simulink model "r2_b8a4x1kf"  (R2012b)
settings: Solver=VariableStepDiscrete  SolverMode=SingleTasking  StartTime=0.0  StopTime=1  RelTol=1e-3
undefined symbols (not defined in the file): fft_stages, n_bits_ants, n_bits_xengs
libraries: xbsIndex_r4 x22142, casper_library_misc x166, xbsReplacements_r4 x24, casper_library_delays x8, xps_library x5, casper_library_communications x4
(part 120 of 178)

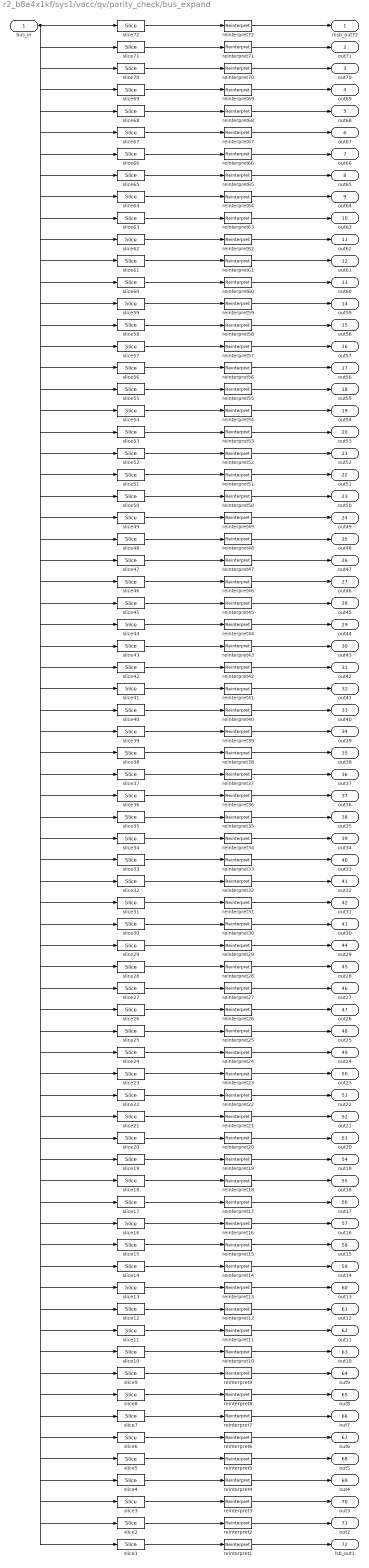
== system r2_b8a4x1kf/sys1/vacc/qv/parity_check/bus_expand ==
  bus_in : Inport
  reinterpret{1..72} (72 alike) : xbsIndex_r4/Reinterpret  force_arith_type=on  arith_type=Unsigned  force_bin_pt=on  bin_pt=0  block_type=reinterpret
  slice1 : xbsIndex_r4/Slice  nbits=1  boolean_output=off  mode=Upper Bit Location + Width  bit1=-71  base1=MSB of Input  bit0=0  base0=LSB of Input  dbl_ovrd=off  block_type=slice
  slice10 : xbsIndex_r4/Slice  nbits=1  boolean_output=off  mode=Upper Bit Location + Width  bit1=-62  base1=MSB of Input  bit0=0  base0=LSB of Input  dbl_ovrd=off  block_type=slice
  slice11 : xbsIndex_r4/Slice  nbits=1  boolean_output=off  mode=Upper Bit Location + Width  bit1=-61  base1=MSB of Input  bit0=0  base0=LSB of Input  dbl_ovrd=off  block_type=slice
  slice12 : xbsIndex_r4/Slice  nbits=1  boolean_output=off  mode=Upper Bit Location + Width  bit1=-60  base1=MSB of Input  bit0=0  base0=LSB of Input  dbl_ovrd=off  block_type=slice
  slice13 : xbsIndex_r4/Slice  nbits=1  boolean_output=off  mode=Upper Bit Location + Width  bit1=-59  base1=MSB of Input  bit0=0  base0=LSB of Input  dbl_ovrd=off  block_type=slice
  slice14 : xbsIndex_r4/Slice  nbits=1  boolean_output=off  mode=Upper Bit Location + Width  bit1=-58  base1=MSB of Input  bit0=0  base0=LSB of Input  dbl_ovrd=off  block_type=slice
  slice15 : xbsIndex_r4/Slice  nbits=1  boolean_output=off  mode=Upper Bit Location + Width  bit1=-57  base1=MSB of Input  bit0=0  base0=LSB of Input  dbl_ovrd=off  block_type=slice
  slice16 : xbsIndex_r4/Slice  nbits=1  boolean_output=off  mode=Upper Bit Location + Width  bit1=-56  base1=MSB of Input  bit0=0  base0=LSB of Input  dbl_ovrd=off  block_type=slice
  slice17 : xbsIndex_r4/Slice  nbits=1  boolean_output=off  mode=Upper Bit Location + Width  bit1=-55  base1=MSB of Input  bit0=0  base0=LSB of Input  dbl_ovrd=off  block_type=slice
  slice18 : xbsIndex_r4/Slice  nbits=1  boolean_output=off  mode=Upper Bit Location + Width  bit1=-54  base1=MSB of Input  bit0=0  base0=LSB of Input  dbl_ovrd=off  block_type=slice
  slice19 : xbsIndex_r4/Slice  nbits=1  boolean_output=off  mode=Upper Bit Location + Width  bit1=-53  base1=MSB of Input  bit0=0  base0=LSB of Input  dbl_ovrd=off  block_type=slice
  slice2 : xbsIndex_r4/Slice  nbits=1  boolean_output=off  mode=Upper Bit Location + Width  bit1=-70  base1=MSB of Input  bit0=0  base0=LSB of Input  dbl_ovrd=off  block_type=slice
  slice20 : xbsIndex_r4/Slice  nbits=1  boolean_output=off  mode=Upper Bit Location + Width  bit1=-52  base1=MSB of Input  bit0=0  base0=LSB of Input  dbl_ovrd=off  block_type=slice
  slice21 : xbsIndex_r4/Slice  nbits=1  boolean_output=off  mode=Upper Bit Location + Width  bit1=-51  base1=MSB of Input  bit0=0  base0=LSB of Input  dbl_ovrd=off  block_type=slice
  slice22 : xbsIndex_r4/Slice  nbits=1  boolean_output=off  mode=Upper Bit Location + Width  bit1=-50  base1=MSB of Input  bit0=0  base0=LSB of Input  dbl_ovrd=off  block_type=slice
  slice23 : xbsIndex_r4/Slice  nbits=1  boolean_output=off  mode=Upper Bit Location + Width  bit1=-49  base1=MSB of Input  bit0=0  base0=LSB of Input  dbl_ovrd=off  block_type=slice
  slice24 : xbsIndex_r4/Slice  nbits=1  boolean_output=off  mode=Upper Bit Location + Width  bit1=-48  base1=MSB of Input  bit0=0  base0=LSB of Input  dbl_ovrd=off  block_type=slice
  slice25 : xbsIndex_r4/Slice  nbits=1  boolean_output=off  mode=Upper Bit Location + Width  bit1=-47  base1=MSB of Input  bit0=0  base0=LSB of Input  dbl_ovrd=off  block_type=slice
  slice26 : xbsIndex_r4/Slice  nbits=1  boolean_output=off  mode=Upper Bit Location + Width  bit1=-46  base1=MSB of Input  bit0=0  base0=LSB of Input  dbl_ovrd=off  block_type=slice
  slice27 : xbsIndex_r4/Slice  nbits=1  boolean_output=off  mode=Upper Bit Location + Width  bit1=-45  base1=MSB of Input  bit0=0  base0=LSB of Input  dbl_ovrd=off  block_type=slice
  slice28 : xbsIndex_r4/Slice  nbits=1  boolean_output=off  mode=Upper Bit Location + Width  bit1=-44  base1=MSB of Input  bit0=0  base0=LSB of Input  dbl_ovrd=off  block_type=slice
  slice29 : xbsIndex_r4/Slice  nbits=1  boolean_output=off  mode=Upper Bit Location + Width  bit1=-43  base1=MSB of Input  bit0=0  base0=LSB of Input  dbl_ovrd=off  block_type=slice
  slice3 : xbsIndex_r4/Slice  nbits=1  boolean_output=off  mode=Upper Bit Location + Width  bit1=-69  base1=MSB of Input  bit0=0  base0=LSB of Input  dbl_ovrd=off  block_type=slice
  slice30 : xbsIndex_r4/Slice  nbits=1  boolean_output=off  mode=Upper Bit Location + Width  bit1=-42  base1=MSB of Input  bit0=0  base0=LSB of Input  dbl_ovrd=off  block_type=slice
  slice31 : xbsIndex_r4/Slice  nbits=1  boolean_output=off  mode=Upper Bit Location + Width  bit1=-41  base1=MSB of Input  bit0=0  base0=LSB of Input  dbl_ovrd=off  block_type=slice
  slice32 : xbsIndex_r4/Slice  nbits=1  boolean_output=off  mode=Upper Bit Location + Width  bit1=-40  base1=MSB of Input  bit0=0  base0=LSB of Input  dbl_ovrd=off  block_type=slice
  slice33 : xbsIndex_r4/Slice  nbits=1  boolean_output=off  mode=Upper Bit Location + Width  bit1=-39  base1=MSB of Input  bit0=0  base0=LSB of Input  dbl_ovrd=off  block_type=slice
  slice34 : xbsIndex_r4/Slice  nbits=1  boolean_output=off  mode=Upper Bit Location + Width  bit1=-38  base1=MSB of Input  bit0=0  base0=LSB of Input  dbl_ovrd=off  block_type=slice
  slice35 : xbsIndex_r4/Slice  nbits=1  boolean_output=off  mode=Upper Bit Location + Width  bit1=-37  base1=MSB of Input  bit0=0  base0=LSB of Input  dbl_ovrd=off  block_type=slice
  slice36 : xbsIndex_r4/Slice  nbits=1  boolean_output=off  mode=Upper Bit Location + Width  bit1=-36  base1=MSB of Input  bit0=0  base0=LSB of Input  dbl_ovrd=off  block_type=slice
  slice37 : xbsIndex_r4/Slice  nbits=1  boolean_output=off  mode=Upper Bit Location + Width  bit1=-35  base1=MSB of Input  bit0=0  base0=LSB of Input  dbl_ovrd=off  block_type=slice
  slice38 : xbsIndex_r4/Slice  nbits=1  boolean_output=off  mode=Upper Bit Location + Width  bit1=-34  base1=MSB of Input  bit0=0  base0=LSB of Input  dbl_ovrd=off  block_type=slice
  slice39 : xbsIndex_r4/Slice  nbits=1  boolean_output=off  mode=Upper Bit Location + Width  bit1=-33  base1=MSB of Input  bit0=0  base0=LSB of Input  dbl_ovrd=off  block_type=slice
  slice4 : xbsIndex_r4/Slice  nbits=1  boolean_output=off  mode=Upper Bit Location + Width  bit1=-68  base1=MSB of Input  bit0=0  base0=LSB of Input  dbl_ovrd=off  block_type=slice
  slice40 : xbsIndex_r4/Slice  nbits=1  boolean_output=off  mode=Upper Bit Location + Width  bit1=-32  base1=MSB of Input  bit0=0  base0=LSB of Input  dbl_ovrd=off  block_type=slice
  slice41 : xbsIndex_r4/Slice  nbits=1  boolean_output=off  mode=Upper Bit Location + Width  bit1=-31  base1=MSB of Input  bit0=0  base0=LSB of Input  dbl_ovrd=off  block_type=slice
  slice42 : xbsIndex_r4/Slice  nbits=1  boolean_output=off  mode=Upper Bit Location + Width  bit1=-30  base1=MSB of Input  bit0=0  base0=LSB of Input  dbl_ovrd=off  block_type=slice
  slice43 : xbsIndex_r4/Slice  nbits=1  boolean_output=off  mode=Upper Bit Location + Width  bit1=-29  base1=MSB of Input  bit0=0  base0=LSB of Input  dbl_ovrd=off  block_type=slice
  slice44 : xbsIndex_r4/Slice  nbits=1  boolean_output=off  mode=Upper Bit Location + Width  bit1=-28  base1=MSB of Input  bit0=0  base0=LSB of Input  dbl_ovrd=off  block_type=slice
  slice45 : xbsIndex_r4/Slice  nbits=1  boolean_output=off  mode=Upper Bit Location + Width  bit1=-27  base1=MSB of Input  bit0=0  base0=LSB of Input  dbl_ovrd=off  block_type=slice
  slice46 : xbsIndex_r4/Slice  nbits=1  boolean_output=off  mode=Upper Bit Location + Width  bit1=-26  base1=MSB of Input  bit0=0  base0=LSB of Input  dbl_ovrd=off  block_type=slice
  slice47 : xbsIndex_r4/Slice  nbits=1  boolean_output=off  mode=Upper Bit Location + Width  bit1=-25  base1=MSB of Input  bit0=0  base0=LSB of Input  dbl_ovrd=off  block_type=slice
  slice48 : xbsIndex_r4/Slice  nbits=1  boolean_output=off  mode=Upper Bit Location + Width  bit1=-24  base1=MSB of Input  bit0=0  base0=LSB of Input  dbl_ovrd=off  block_type=slice
  slice49 : xbsIndex_r4/Slice  nbits=1  boolean_output=off  mode=Upper Bit Location + Width  bit1=-23  base1=MSB of Input  bit0=0  base0=LSB of Input  dbl_ovrd=off  block_type=slice
  slice5 : xbsIndex_r4/Slice  nbits=1  boolean_output=off  mode=Upper Bit Location + Width  bit1=-67  base1=MSB of Input  bit0=0  base0=LSB of Input  dbl_ovrd=off  block_type=slice
  slice50 : xbsIndex_r4/Slice  nbits=1  boolean_output=off  mode=Upper Bit Location + Width  bit1=-22  base1=MSB of Input  bit0=0  base0=LSB of Input  dbl_ovrd=off  block_type=slice
  slice51 : xbsIndex_r4/Slice  nbits=1  boolean_output=off  mode=Upper Bit Location + Width  bit1=-21  base1=MSB of Input  bit0=0  base0=LSB of Input  dbl_ovrd=off  block_type=slice
  slice52 : xbsIndex_r4/Slice  nbits=1  boolean_output=off  mode=Upper Bit Location + Width  bit1=-20  base1=MSB of Input  bit0=0  base0=LSB of Input  dbl_ovrd=off  block_type=slice
  slice53 : xbsIndex_r4/Slice  nbits=1  boolean_output=off  mode=Upper Bit Location + Width  bit1=-19  base1=MSB of Input  bit0=0  base0=LSB of Input  dbl_ovrd=off  block_type=slice
  slice54 : xbsIndex_r4/Slice  nbits=1  boolean_output=off  mode=Upper Bit Location + Width  bit1=-18  base1=MSB of Input  bit0=0  base0=LSB of Input  dbl_ovrd=off  block_type=slice
  slice55 : xbsIndex_r4/Slice  nbits=1  boolean_output=off  mode=Upper Bit Location + Width  bit1=-17  base1=MSB of Input  bit0=0  base0=LSB of Input  dbl_ovrd=off  block_type=slice
  slice56 : xbsIndex_r4/Slice  nbits=1  boolean_output=off  mode=Upper Bit Location + Width  bit1=-16  base1=MSB of Input  bit0=0  base0=LSB of Input  dbl_ovrd=off  block_type=slice
  slice57 : xbsIndex_r4/Slice  nbits=1  boolean_output=off  mode=Upper Bit Location + Width  bit1=-15  base1=MSB of Input  bit0=0  base0=LSB of Input  dbl_ovrd=off  block_type=slice
  slice58 : xbsIndex_r4/Slice  nbits=1  boolean_output=off  mode=Upper Bit Location + Width  bit1=-14  base1=MSB of Input  bit0=0  base0=LSB of Input  dbl_ovrd=off  block_type=slice
  slice59 : xbsIndex_r4/Slice  nbits=1  boolean_output=off  mode=Upper Bit Location + Width  bit1=-13  base1=MSB of Input  bit0=0  base0=LSB of Input  dbl_ovrd=off  block_type=slice
  slice6 : xbsIndex_r4/Slice  nbits=1  boolean_output=off  mode=Upper Bit Location + Width  bit1=-66  base1=MSB of Input  bit0=0  base0=LSB of Input  dbl_ovrd=off  block_type=slice
  slice60 : xbsIndex_r4/Slice  nbits=1  boolean_output=off  mode=Upper Bit Location + Width  bit1=-12  base1=MSB of Input  bit0=0  base0=LSB of Input  dbl_ovrd=off  block_type=slice
  slice61 : xbsIndex_r4/Slice  nbits=1  boolean_output=off  mode=Upper Bit Location + Width  bit1=-11  base1=MSB of Input  bit0=0  base0=LSB of Input  dbl_ovrd=off  block_type=slice
  slice62 : xbsIndex_r4/Slice  nbits=1  boolean_output=off  mode=Upper Bit Location + Width  bit1=-10  base1=MSB of Input  bit0=0  base0=LSB of Input  dbl_ovrd=off  block_type=slice
  slice63 : xbsIndex_r4/Slice  nbits=1  boolean_output=off  mode=Upper Bit Location + Width  bit1=-9  base1=MSB of Input  bit0=0  base0=LSB of Input  dbl_ovrd=off  block_type=slice
  slice64 : xbsIndex_r4/Slice  nbits=1  boolean_output=off  mode=Upper Bit Location + Width  bit1=-8  base1=MSB of Input  bit0=0  base0=LSB of Input  dbl_ovrd=off  block_type=slice
  slice65 : xbsIndex_r4/Slice  nbits=1  boolean_output=off  mode=Upper Bit Location + Width  bit1=-7  base1=MSB of Input  bit0=0  base0=LSB of Input  dbl_ovrd=off  block_type=slice
  slice66 : xbsIndex_r4/Slice  nbits=1  boolean_output=off  mode=Upper Bit Location + Width  bit1=-6  base1=MSB of Input  bit0=0  base0=LSB of Input  dbl_ovrd=off  block_type=slice
  slice67 : xbsIndex_r4/Slice  nbits=1  boolean_output=off  mode=Upper Bit Location + Width  bit1=-5  base1=MSB of Input  bit0=0  base0=LSB of Input  dbl_ovrd=off  block_type=slice
  slice68 : xbsIndex_r4/Slice  nbits=1  boolean_output=off  mode=Upper Bit Location + Width  bit1=-4  base1=MSB of Input  bit0=0  base0=LSB of Input  dbl_ovrd=off  block_type=slice
  slice69 : xbsIndex_r4/Slice  nbits=1  boolean_output=off  mode=Upper Bit Location + Width  bit1=-3  base1=MSB of Input  bit0=0  base0=LSB of Input  dbl_ovrd=off  block_type=slice
  slice7 : xbsIndex_r4/Slice  nbits=1  boolean_output=off  mode=Upper Bit Location + Width  bit1=-65  base1=MSB of Input  bit0=0  base0=LSB of Input  dbl_ovrd=off  block_type=slice
  slice70 : xbsIndex_r4/Slice  nbits=1  boolean_output=off  mode=Upper Bit Location + Width  bit1=-2  base1=MSB of Input  bit0=0  base0=LSB of Input  dbl_ovrd=off  block_type=slice
  slice71 : xbsIndex_r4/Slice  nbits=1  boolean_output=off  mode=Upper Bit Location + Width  bit1=-1  base1=MSB of Input  bit0=0  base0=LSB of Input  dbl_ovrd=off  block_type=slice
  slice72 : xbsIndex_r4/Slice  nbits=1  boolean_output=off  mode=Upper Bit Location + Width  bit1=0  base1=MSB of Input  bit0=0  base0=LSB of Input  dbl_ovrd=off  block_type=slice
  slice8 : xbsIndex_r4/Slice  nbits=1  boolean_output=off  mode=Upper Bit Location + Width  bit1=-64  base1=MSB of Input  bit0=0  base0=LSB of Input  dbl_ovrd=off  block_type=slice
  slice9 : xbsIndex_r4/Slice  nbits=1  boolean_output=off  mode=Upper Bit Location + Width  bit1=-63  base1=MSB of Input  bit0=0  base0=LSB of Input  dbl_ovrd=off  block_type=slice
  msb_out72 : Outport
  out71 : Outport  Port=2
  out70 : Outport  Port=3
  out69 : Outport  Port=4
  out68 : Outport  Port=5
  out67 : Outport  Port=6
  out66 : Outport  Port=7
  out65 : Outport  Port=8
  out64 : Outport  Port=9
  out63 : Outport  Port=10
  out62 : Outport  Port=11
  out61 : Outport  Port=12
  out60 : Outport  Port=13
  out59 : Outport  Port=14
  out58 : Outport  Port=15
  out57 : Outport  Port=16
  out56 : Outport  Port=17
  out55 : Outport  Port=18
  out54 : Outport  Port=19
  out53 : Outport  Port=20
  out52 : Outport  Port=21
  out51 : Outport  Port=22
  out50 : Outport  Port=23
  out49 : Outport  Port=24
  out48 : Outport  Port=25
  out47 : Outport  Port=26
  out46 : Outport  Port=27
  out45 : Outport  Port=28
  out44 : Outport  Port=29
  out43 : Outport  Port=30
  out42 : Outport  Port=31
  out41 : Outport  Port=32
  out40 : Outport  Port=33
  out39 : Outport  Port=34
  out38 : Outport  Port=35
  out37 : Outport  Port=36
  out36 : Outport  Port=37
  out35 : Outport  Port=38
  out34 : Outport  Port=39
  out33 : Outport  Port=40
  out32 : Outport  Port=41
  out31 : Outport  Port=42
  out30 : Outport  Port=43
  out29 : Outport  Port=44
  out28 : Outport  Port=45
  out27 : Outport  Port=46
  out26 : Outport  Port=47
  out25 : Outport  Port=48
  out24 : Outport  Port=49
  out23 : Outport  Port=50
  out22 : Outport  Port=51
  out21 : Outport  Port=52
  out20 : Outport  Port=53
  out19 : Outport  Port=54
  out18 : Outport  Port=55
  out17 : Outport  Port=56
  out16 : Outport  Port=57
  out15 : Outport  Port=58
  out14 : Outport  Port=59
  out13 : Outport  Port=60
  out12 : Outport  Port=61
  out11 : Outport  Port=62
  out10 : Outport  Port=63
  out9 : Outport  Port=64
  out8 : Outport  Port=65
  out7 : Outport  Port=66
  out6 : Outport  Port=67
  out5 : Outport  Port=68
  out4 : Outport  Port=69
  out3 : Outport  Port=70
  out2 : Outport  Port=71
  lsb_out1 : Outport  Port=72
  wires:
  reinterpret1/1 -> lsb_out1/1
  slice1/1 -> reinterpret1/1
  reinterpret2/1 -> out2/1
  slice2/1 -> reinterpret2/1
  reinterpret3/1 -> out3/1
  slice3/1 -> reinterpret3/1
  reinterpret4/1 -> out4/1
  slice4/1 -> reinterpret4/1
  reinterpret5/1 -> out5/1
  slice5/1 -> reinterpret5/1
  reinterpret6/1 -> out6/1
  slice6/1 -> reinterpret6/1
  reinterpret7/1 -> out7/1
  slice7/1 -> reinterpret7/1
  reinterpret8/1 -> out8/1
  slice8/1 -> reinterpret8/1
  reinterpret9/1 -> out9/1
  slice9/1 -> reinterpret9/1
  reinterpret10/1 -> out10/1
  slice10/1 -> reinterpret10/1
  reinterpret11/1 -> out11/1
  slice11/1 -> reinterpret11/1
  reinterpret12/1 -> out12/1
  slice12/1 -> reinterpret12/1
  reinterpret13/1 -> out13/1
  slice13/1 -> reinterpret13/1
  reinterpret14/1 -> out14/1
  slice14/1 -> reinterpret14/1
  reinterpret15/1 -> out15/1
  slice15/1 -> reinterpret15/1
  reinterpret16/1 -> out16/1
  slice16/1 -> reinterpret16/1
  reinterpret17/1 -> out17/1
  slice17/1 -> reinterpret17/1
  reinterpret18/1 -> out18/1
  slice18/1 -> reinterpret18/1
  reinterpret19/1 -> out19/1
  slice19/1 -> reinterpret19/1
  reinterpret20/1 -> out20/1
  slice20/1 -> reinterpret20/1
  reinterpret21/1 -> out21/1
  slice21/1 -> reinterpret21/1
  reinterpret22/1 -> out22/1
  slice22/1 -> reinterpret22/1
  reinterpret23/1 -> out23/1
  slice23/1 -> reinterpret23/1
  reinterpret24/1 -> out24/1
  slice24/1 -> reinterpret24/1
  reinterpret25/1 -> out25/1
  slice25/1 -> reinterpret25/1
  reinterpret26/1 -> out26/1
  slice26/1 -> reinterpret26/1
  reinterpret27/1 -> out27/1
  slice27/1 -> reinterpret27/1
  reinterpret28/1 -> out28/1
  slice28/1 -> reinterpret28/1
  reinterpret29/1 -> out29/1
  slice29/1 -> reinterpret29/1
  reinterpret30/1 -> out30/1
  slice30/1 -> reinterpret30/1
  reinterpret31/1 -> out31/1
  slice31/1 -> reinterpret31/1
  reinterpret32/1 -> out32/1
  slice32/1 -> reinterpret32/1
  reinterpret33/1 -> out33/1
  slice33/1 -> reinterpret33/1
  reinterpret34/1 -> out34/1
  slice34/1 -> reinterpret34/1
  reinterpret35/1 -> out35/1
  slice35/1 -> reinterpret35/1
  reinterpret36/1 -> out36/1
  slice36/1 -> reinterpret36/1
  reinterpret37/1 -> out37/1
  slice37/1 -> reinterpret37/1
  reinterpret38/1 -> out38/1
  slice38/1 -> reinterpret38/1
  reinterpret39/1 -> out39/1
  slice39/1 -> reinterpret39/1
  reinterpret40/1 -> out40/1
  slice40/1 -> reinterpret40/1
  reinterpret41/1 -> out41/1
  slice41/1 -> reinterpret41/1
  reinterpret42/1 -> out42/1
  slice42/1 -> reinterpret42/1
  reinterpret43/1 -> out43/1
  slice43/1 -> reinterpret43/1
  reinterpret44/1 -> out44/1
  slice44/1 -> reinterpret44/1
  reinterpret45/1 -> out45/1
  slice45/1 -> reinterpret45/1
  reinterpret46/1 -> out46/1
  slice46/1 -> reinterpret46/1
  reinterpret47/1 -> out47/1
  slice47/1 -> reinterpret47/1
  reinterpret48/1 -> out48/1
  slice48/1 -> reinterpret48/1
  reinterpret49/1 -> out49/1
  slice49/1 -> reinterpret49/1
  reinterpret50/1 -> out50/1
  slice50/1 -> reinterpret50/1
  reinterpret51/1 -> out51/1
  slice51/1 -> reinterpret51/1
  reinterpret52/1 -> out52/1
  slice52/1 -> reinterpret52/1
  reinterpret53/1 -> out53/1
  slice53/1 -> reinterpret53/1
  reinterpret54/1 -> out54/1
  slice54/1 -> reinterpret54/1
  reinterpret55/1 -> out55/1
  slice55/1 -> reinterpret55/1
  reinterpret56/1 -> out56/1
  slice56/1 -> reinterpret56/1
  reinterpret57/1 -> out57/1
  slice57/1 -> reinterpret57/1
  reinterpret58/1 -> out58/1
  slice58/1 -> reinterpret58/1
  reinterpret59/1 -> out59/1
  slice59/1 -> reinterpret59/1
  reinterpret60/1 -> out60/1
  slice60/1 -> reinterpret60/1
  reinterpret61/1 -> out61/1
  slice61/1 -> reinterpret61/1
  reinterpret62/1 -> out62/1
  slice62/1 -> reinterpret62/1
  reinterpret63/1 -> out63/1
  slice63/1 -> reinterpret63/1
  reinterpret64/1 -> out64/1
  slice64/1 -> reinterpret64/1
  reinterpret65/1 -> out65/1
  slice65/1 -> reinterpret65/1
  reinterpret66/1 -> out66/1
  slice66/1 -> reinterpret66/1
  reinterpret67/1 -> out67/1
  slice67/1 -> reinterpret67/1
  reinterpret68/1 -> out68/1
  slice68/1 -> reinterpret68/1
  reinterpret69/1 -> out69/1
  slice69/1 -> reinterpret69/1
  reinterpret70/1 -> out70/1
  slice70/1 -> reinterpret70/1
  reinterpret71/1 -> out71/1
  slice71/1 -> reinterpret71/1
  reinterpret72/1 -> msb_out72/1
  slice72/1 -> reinterpret72/1
  bus_in/1 -> slice1/1, slice2/1, slice3/1, slice4/1, slice5/1, slice6/1, slice7/1, slice8/1, slice9/1, slice10/1, slice11/1, slice12/1, slice13/1, slice14/1, slice15/1, slice16/1, slice17/1, slice18/1, slice19/1, slice20/1, slice21/1, slice22/1, slice23/1, slice24/1, slice25/1, slice26/1, slice27/1, slice28/1, slice29/1, slice30/1, slice31/1, slice32/1, slice33/1, slice34/1, slice35/1, slice36/1, slice37/1, slice38/1, slice39/1, slice40/1, slice41/1, slice42/1, slice43/1, slice44/1, slice45/1, slice46/1, slice47/1, slice48/1, slice49/1, slice50/1, slice51/1, slice52/1, slice53/1, slice54/1, slice55/1, slice56/1, slice57/1, slice58/1, slice59/1, slice60/1, slice61/1, slice62/1, slice63/1, slice64/1, slice65/1, slice66/1, slice67/1, slice68/1, slice69/1, slice70/1, slice71/1, slice72/1

== system r2_b8a4x1kf/sys1/vacc/qv/parity_insertion/bus_expand ==
  bus_in : Inport
  reinterpret{1..71} (71 alike) : xbsIndex_r4/Reinterpret  force_arith_type=on  arith_type=Unsigned  force_bin_pt=on  bin_pt=0  block_type=reinterpret
  slice1 : xbsIndex_r4/Slice  nbits=1  boolean_output=off  mode=Upper Bit Location + Width  bit1=-70  base1=MSB of Input  bit0=0  base0=LSB of Input  dbl_ovrd=off  block_type=slice
  slice10 : xbsIndex_r4/Slice  nbits=1  boolean_output=off  mode=Upper Bit Location + Width  bit1=-61  base1=MSB of Input  bit0=0  base0=LSB of Input  dbl_ovrd=off  block_type=slice
  slice11 : xbsIndex_r4/Slice  nbits=1  boolean_output=off  mode=Upper Bit Location + Width  bit1=-60  base1=MSB of Input  bit0=0  base0=LSB of Input  dbl_ovrd=off  block_type=slice
  slice12 : xbsIndex_r4/Slice  nbits=1  boolean_output=off  mode=Upper Bit Location + Width  bit1=-59  base1=MSB of Input  bit0=0  base0=LSB of Input  dbl_ovrd=off  block_type=slice
  slice13 : xbsIndex_r4/Slice  nbits=1  boolean_output=off  mode=Upper Bit Location + Width  bit1=-58  base1=MSB of Input  bit0=0  base0=LSB of Input  dbl_ovrd=off  block_type=slice
  slice14 : xbsIndex_r4/Slice  nbits=1  boolean_output=off  mode=Upper Bit Location + Width  bit1=-57  base1=MSB of Input  bit0=0  base0=LSB of Input  dbl_ovrd=off  block_type=slice
  slice15 : xbsIndex_r4/Slice  nbits=1  boolean_output=off  mode=Upper Bit Location + Width  bit1=-56  base1=MSB of Input  bit0=0  base0=LSB of Input  dbl_ovrd=off  block_type=slice
  slice16 : xbsIndex_r4/Slice  nbits=1  boolean_output=off  mode=Upper Bit Location + Width  bit1=-55  base1=MSB of Input  bit0=0  base0=LSB of Input  dbl_ovrd=off  block_type=slice
  slice17 : xbsIndex_r4/Slice  nbits=1  boolean_output=off  mode=Upper Bit Location + Width  bit1=-54  base1=MSB of Input  bit0=0  base0=LSB of Input  dbl_ovrd=off  block_type=slice
  slice18 : xbsIndex_r4/Slice  nbits=1  boolean_output=off  mode=Upper Bit Location + Width  bit1=-53  base1=MSB of Input  bit0=0  base0=LSB of Input  dbl_ovrd=off  block_type=slice
  slice19 : xbsIndex_r4/Slice  nbits=1  boolean_output=off  mode=Upper Bit Location + Width  bit1=-52  base1=MSB of Input  bit0=0  base0=LSB of Input  dbl_ovrd=off  block_type=slice
  slice2 : xbsIndex_r4/Slice  nbits=1  boolean_output=off  mode=Upper Bit Location + Width  bit1=-69  base1=MSB of Input  bit0=0  base0=LSB of Input  dbl_ovrd=off  block_type=slice
  slice20 : xbsIndex_r4/Slice  nbits=1  boolean_output=off  mode=Upper Bit Location + Width  bit1=-51  base1=MSB of Input  bit0=0  base0=LSB of Input  dbl_ovrd=off  block_type=slice
  slice21 : xbsIndex_r4/Slice  nbits=1  boolean_output=off  mode=Upper Bit Location + Width  bit1=-50  base1=MSB of Input  bit0=0  base0=LSB of Input  dbl_ovrd=off  block_type=slice
  slice22 : xbsIndex_r4/Slice  nbits=1  boolean_output=off  mode=Upper Bit Location + Width  bit1=-49  base1=MSB of Input  bit0=0  base0=LSB of Input  dbl_ovrd=off  block_type=slice
  slice23 : xbsIndex_r4/Slice  nbits=1  boolean_output=off  mode=Upper Bit Location + Width  bit1=-48  base1=MSB of Input  bit0=0  base0=LSB of Input  dbl_ovrd=off  block_type=slice
  slice24 : xbsIndex_r4/Slice  nbits=1  boolean_output=off  mode=Upper Bit Location + Width  bit1=-47  base1=MSB of Input  bit0=0  base0=LSB of Input  dbl_ovrd=off  block_type=slice
  slice25 : xbsIndex_r4/Slice  nbits=1  boolean_output=off  mode=Upper Bit Location + Width  bit1=-46  base1=MSB of Input  bit0=0  base0=LSB of Input  dbl_ovrd=off  block_type=slice
  slice26 : xbsIndex_r4/Slice  nbits=1  boolean_output=off  mode=Upper Bit Location + Width  bit1=-45  base1=MSB of Input  bit0=0  base0=LSB of Input  dbl_ovrd=off  block_type=slice
  slice27 : xbsIndex_r4/Slice  nbits=1  boolean_output=off  mode=Upper Bit Location + Width  bit1=-44  base1=MSB of Input  bit0=0  base0=LSB of Input  dbl_ovrd=off  block_type=slice
  slice28 : xbsIndex_r4/Slice  nbits=1  boolean_output=off  mode=Upper Bit Location + Width  bit1=-43  base1=MSB of Input  bit0=0  base0=LSB of Input  dbl_ovrd=off  block_type=slice
  slice29 : xbsIndex_r4/Slice  nbits=1  boolean_output=off  mode=Upper Bit Location + Width  bit1=-42  base1=MSB of Input  bit0=0  base0=LSB of Input  dbl_ovrd=off  block_type=slice
  slice3 : xbsIndex_r4/Slice  nbits=1  boolean_output=off  mode=Upper Bit Location + Width  bit1=-68  base1=MSB of Input  bit0=0  base0=LSB of Input  dbl_ovrd=off  block_type=slice
  slice30 : xbsIndex_r4/Slice  nbits=1  boolean_output=off  mode=Upper Bit Location + Width  bit1=-41  base1=MSB of Input  bit0=0  base0=LSB of Input  dbl_ovrd=off  block_type=slice
  slice31 : xbsIndex_r4/Slice  nbits=1  boolean_output=off  mode=Upper Bit Location + Width  bit1=-40  base1=MSB of Input  bit0=0  base0=LSB of Input  dbl_ovrd=off  block_type=slice
  slice32 : xbsIndex_r4/Slice  nbits=1  boolean_output=off  mode=Upper Bit Location + Width  bit1=-39  base1=MSB of Input  bit0=0  base0=LSB of Input  dbl_ovrd=off  block_type=slice
  slice33 : xbsIndex_r4/Slice  nbits=1  boolean_output=off  mode=Upper Bit Location + Width  bit1=-38  base1=MSB of Input  bit0=0  base0=LSB of Input  dbl_ovrd=off  block_type=slice
  slice34 : xbsIndex_r4/Slice  nbits=1  boolean_output=off  mode=Upper Bit Location + Width  bit1=-37  base1=MSB of Input  bit0=0  base0=LSB of Input  dbl_ovrd=off  block_type=slice
  slice35 : xbsIndex_r4/Slice  nbits=1  boolean_output=off  mode=Upper Bit Location + Width  bit1=-36  base1=MSB of Input  bit0=0  base0=LSB of Input  dbl_ovrd=off  block_type=slice
  slice36 : xbsIndex_r4/Slice  nbits=1  boolean_output=off  mode=Upper Bit Location + Width  bit1=-35  base1=MSB of Input  bit0=0  base0=LSB of Input  dbl_ovrd=off  block_type=slice
  slice37 : xbsIndex_r4/Slice  nbits=1  boolean_output=off  mode=Upper Bit Location + Width  bit1=-34  base1=MSB of Input  bit0=0  base0=LSB of Input  dbl_ovrd=off  block_type=slice
  slice38 : xbsIndex_r4/Slice  nbits=1  boolean_output=off  mode=Upper Bit Location + Width  bit1=-33  base1=MSB of Input  bit0=0  base0=LSB of Input  dbl_ovrd=off  block_type=slice
  slice39 : xbsIndex_r4/Slice  nbits=1  boolean_output=off  mode=Upper Bit Location + Width  bit1=-32  base1=MSB of Input  bit0=0  base0=LSB of Input  dbl_ovrd=off  block_type=slice
  slice4 : xbsIndex_r4/Slice  nbits=1  boolean_output=off  mode=Upper Bit Location + Width  bit1=-67  base1=MSB of Input  bit0=0  base0=LSB of Input  dbl_ovrd=off  block_type=slice
  slice40 : xbsIndex_r4/Slice  nbits=1  boolean_output=off  mode=Upper Bit Location + Width  bit1=-31  base1=MSB of Input  bit0=0  base0=LSB of Input  dbl_ovrd=off  block_type=slice
  slice41 : xbsIndex_r4/Slice  nbits=1  boolean_output=off  mode=Upper Bit Location + Width  bit1=-30  base1=MSB of Input  bit0=0  base0=LSB of Input  dbl_ovrd=off  block_type=slice
  slice42 : xbsIndex_r4/Slice  nbits=1  boolean_output=off  mode=Upper Bit Location + Width  bit1=-29  base1=MSB of Input  bit0=0  base0=LSB of Input  dbl_ovrd=off  block_type=slice
  slice43 : xbsIndex_r4/Slice  nbits=1  boolean_output=off  mode=Upper Bit Location + Width  bit1=-28  base1=MSB of Input  bit0=0  base0=LSB of Input  dbl_ovrd=off  block_type=slice
  slice44 : xbsIndex_r4/Slice  nbits=1  boolean_output=off  mode=Upper Bit Location + Width  bit1=-27  base1=MSB of Input  bit0=0  base0=LSB of Input  dbl_ovrd=off  block_type=slice
  slice45 : xbsIndex_r4/Slice  nbits=1  boolean_output=off  mode=Upper Bit Location + Width  bit1=-26  base1=MSB of Input  bit0=0  base0=LSB of Input  dbl_ovrd=off  block_type=slice
  slice46 : xbsIndex_r4/Slice  nbits=1  boolean_output=off  mode=Upper Bit Location + Width  bit1=-25  base1=MSB of Input  bit0=0  base0=LSB of Input  dbl_ovrd=off  block_type=slice
  slice47 : xbsIndex_r4/Slice  nbits=1  boolean_output=off  mode=Upper Bit Location + Width  bit1=-24  base1=MSB of Input  bit0=0  base0=LSB of Input  dbl_ovrd=off  block_type=slice
  slice48 : xbsIndex_r4/Slice  nbits=1  boolean_output=off  mode=Upper Bit Location + Width  bit1=-23  base1=MSB of Input  bit0=0  base0=LSB of Input  dbl_ovrd=off  block_type=slice
  slice49 : xbsIndex_r4/Slice  nbits=1  boolean_output=off  mode=Upper Bit Location + Width  bit1=-22  base1=MSB of Input  bit0=0  base0=LSB of Input  dbl_ovrd=off  block_type=slice
  slice5 : xbsIndex_r4/Slice  nbits=1  boolean_output=off  mode=Upper Bit Location + Width  bit1=-66  base1=MSB of Input  bit0=0  base0=LSB of Input  dbl_ovrd=off  block_type=slice
  slice50 : xbsIndex_r4/Slice  nbits=1  boolean_output=off  mode=Upper Bit Location + Width  bit1=-21  base1=MSB of Input  bit0=0  base0=LSB of Input  dbl_ovrd=off  block_type=slice
  slice51 : xbsIndex_r4/Slice  nbits=1  boolean_output=off  mode=Upper Bit Location + Width  bit1=-20  base1=MSB of Input  bit0=0  base0=LSB of Input  dbl_ovrd=off  block_type=slice
  slice52 : xbsIndex_r4/Slice  nbits=1  boolean_output=off  mode=Upper Bit Location + Width  bit1=-19  base1=MSB of Input  bit0=0  base0=LSB of Input  dbl_ovrd=off  block_type=slice
  slice53 : xbsIndex_r4/Slice  nbits=1  boolean_output=off  mode=Upper Bit Location + Width  bit1=-18  base1=MSB of Input  bit0=0  base0=LSB of Input  dbl_ovrd=off  block_type=slice
  slice54 : xbsIndex_r4/Slice  nbits=1  boolean_output=off  mode=Upper Bit Location + Width  bit1=-17  base1=MSB of Input  bit0=0  base0=LSB of Input  dbl_ovrd=off  block_type=slice
  slice55 : xbsIndex_r4/Slice  nbits=1  boolean_output=off  mode=Upper Bit Location + Width  bit1=-16  base1=MSB of Input  bit0=0  base0=LSB of Input  dbl_ovrd=off  block_type=slice
  slice56 : xbsIndex_r4/Slice  nbits=1  boolean_output=off  mode=Upper Bit Location + Width  bit1=-15  base1=MSB of Input  bit0=0  base0=LSB of Input  dbl_ovrd=off  block_type=slice
  slice57 : xbsIndex_r4/Slice  nbits=1  boolean_output=off  mode=Upper Bit Location + Width  bit1=-14  base1=MSB of Input  bit0=0  base0=LSB of Input  dbl_ovrd=off  block_type=slice
  slice58 : xbsIndex_r4/Slice  nbits=1  boolean_output=off  mode=Upper Bit Location + Width  bit1=-13  base1=MSB of Input  bit0=0  base0=LSB of Input  dbl_ovrd=off  block_type=slice
  slice59 : xbsIndex_r4/Slice  nbits=1  boolean_output=off  mode=Upper Bit Location + Width  bit1=-12  base1=MSB of Input  bit0=0  base0=LSB of Input  dbl_ovrd=off  block_type=slice
  slice6 : xbsIndex_r4/Slice  nbits=1  boolean_output=off  mode=Upper Bit Location + Width  bit1=-65  base1=MSB of Input  bit0=0  base0=LSB of Input  dbl_ovrd=off  block_type=slice
  slice60 : xbsIndex_r4/Slice  nbits=1  boolean_output=off  mode=Upper Bit Location + Width  bit1=-11  base1=MSB of Input  bit0=0  base0=LSB of Input  dbl_ovrd=off  block_type=slice
  slice61 : xbsIndex_r4/Slice  nbits=1  boolean_output=off  mode=Upper Bit Location + Width  bit1=-10  base1=MSB of Input  bit0=0  base0=LSB of Input  dbl_ovrd=off  block_type=slice
  slice62 : xbsIndex_r4/Slice  nbits=1  boolean_output=off  mode=Upper Bit Location + Width  bit1=-9  base1=MSB of Input  bit0=0  base0=LSB of Input  dbl_ovrd=off  block_type=slice
  slice63 : xbsIndex_r4/Slice  nbits=1  boolean_output=off  mode=Upper Bit Location + Width  bit1=-8  base1=MSB of Input  bit0=0  base0=LSB of Input  dbl_ovrd=off  block_type=slice
  slice64 : xbsIndex_r4/Slice  nbits=1  boolean_output=off  mode=Upper Bit Location + Width  bit1=-7  base1=MSB of Input  bit0=0  base0=LSB of Input  dbl_ovrd=off  block_type=slice
  slice65 : xbsIndex_r4/Slice  nbits=1  boolean_output=off  mode=Upper Bit Location + Width  bit1=-6  base1=MSB of Input  bit0=0  base0=LSB of Input  dbl_ovrd=off  block_type=slice
  slice66 : xbsIndex_r4/Slice  nbits=1  boolean_output=off  mode=Upper Bit Location + Width  bit1=-5  base1=MSB of Input  bit0=0  base0=LSB of Input  dbl_ovrd=off  block_type=slice
  slice67 : xbsIndex_r4/Slice  nbits=1  boolean_output=off  mode=Upper Bit Location + Width  bit1=-4  base1=MSB of Input  bit0=0  base0=LSB of Input  dbl_ovrd=off  block_type=slice
  slice68 : xbsIndex_r4/Slice  nbits=1  boolean_output=off  mode=Upper Bit Location + Width  bit1=-3  base1=MSB of Input  bit0=0  base0=LSB of Input  dbl_ovrd=off  block_type=slice
  slice69 : xbsIndex_r4/Slice  nbits=1  boolean_output=off  mode=Upper Bit Location + Width  bit1=-2  base1=MSB of Input  bit0=0  base0=LSB of Input  dbl_ovrd=off  block_type=slice
  slice7 : xbsIndex_r4/Slice  nbits=1  boolean_output=off  mode=Upper Bit Location + Width  bit1=-64  base1=MSB of Input  bit0=0  base0=LSB of Input  dbl_ovrd=off  block_type=slice
  slice70 : xbsIndex_r4/Slice  nbits=1  boolean_output=off  mode=Upper Bit Location + Width  bit1=-1  base1=MSB of Input  bit0=0  base0=LSB of Input  dbl_ovrd=off  block_type=slice
  slice71 : xbsIndex_r4/Slice  nbits=1  boolean_output=off  mode=Upper Bit Location + Width  bit1=0  base1=MSB of Input  bit0=0  base0=LSB of Input  dbl_ovrd=off  block_type=slice
  slice8 : xbsIndex_r4/Slice  nbits=1  boolean_output=off  mode=Upper Bit Location + Width  bit1=-63  base1=MSB of Input  bit0=0  base0=LSB of Input  dbl_ovrd=off  block_type=slice
  slice9 : xbsIndex_r4/Slice  nbits=1  boolean_output=off  mode=Upper Bit Location + Width  bit1=-62  base1=MSB of Input  bit0=0  base0=LSB of Input  dbl_ovrd=off  block_type=slice
  msb_out71 : Outport
  out70 : Outport  Port=2
  out69 : Outport  Port=3
  out68 : Outport  Port=4
  out67 : Outport  Port=5
  out66 : Outport  Port=6
  out65 : Outport  Port=7
  out64 : Outport  Port=8
  out63 : Outport  Port=9
  out62 : Outport  Port=10
  out61 : Outport  Port=11
  out60 : Outport  Port=12
  out59 : Outport  Port=13
  out58 : Outport  Port=14
  out57 : Outport  Port=15
  out56 : Outport  Port=16
  out55 : Outport  Port=17
  out54 : Outport  Port=18
  out53 : Outport  Port=19
  out52 : Outport  Port=20
  out51 : Outport  Port=21
  out50 : Outport  Port=22
  out49 : Outport  Port=23
  out48 : Outport  Port=24
  out47 : Outport  Port=25
  out46 : Outport  Port=26
  out45 : Outport  Port=27
  out44 : Outport  Port=28
  out43 : Outport  Port=29
  out42 : Outport  Port=30
  out41 : Outport  Port=31
  out40 : Outport  Port=32
  out39 : Outport  Port=33
  out38 : Outport  Port=34
  out37 : Outport  Port=35
  out36 : Outport  Port=36
  out35 : Outport  Port=37
  out34 : Outport  Port=38
  out33 : Outport  Port=39
  out32 : Outport  Port=40
  out31 : Outport  Port=41
  out30 : Outport  Port=42
  out29 : Outport  Port=43
  out28 : Outport  Port=44
  out27 : Outport  Port=45
  out26 : Outport  Port=46
  out25 : Outport  Port=47
  out24 : Outport  Port=48
  out23 : Outport  Port=49
  out22 : Outport  Port=50
  out21 : Outport  Port=51
  out20 : Outport  Port=52
  out19 : Outport  Port=53
  out18 : Outport  Port=54
  out17 : Outport  Port=55
  out16 : Outport  Port=56
  out15 : Outport  Port=57
  out14 : Outport  Port=58
  out13 : Outport  Port=59
  out12 : Outport  Port=60
  out11 : Outport  Port=61
  out10 : Outport  Port=62
  out9 : Outport  Port=63
  out8 : Outport  Port=64
  out7 : Outport  Port=65
  out6 : Outport  Port=66
  out5 : Outport  Port=67
  out4 : Outport  Port=68
  out3 : Outport  Port=69
  out2 : Outport  Port=70
  lsb_out1 : Outport  Port=71
  wires:
  reinterpret1/1 -> lsb_out1/1
  slice1/1 -> reinterpret1/1
  reinterpret2/1 -> out2/1
  slice2/1 -> reinterpret2/1
  reinterpret3/1 -> out3/1
  slice3/1 -> reinterpret3/1
  reinterpret4/1 -> out4/1
  slice4/1 -> reinterpret4/1
  reinterpret5/1 -> out5/1
  slice5/1 -> reinterpret5/1
  reinterpret6/1 -> out6/1
  slice6/1 -> reinterpret6/1
  reinterpret7/1 -> out7/1
  slice7/1 -> reinterpret7/1
  reinterpret8/1 -> out8/1
  slice8/1 -> reinterpret8/1
  reinterpret9/1 -> out9/1
  slice9/1 -> reinterpret9/1
  reinterpret10/1 -> out10/1
  slice10/1 -> reinterpret10/1
  reinterpret11/1 -> out11/1
  slice11/1 -> reinterpret11/1
  reinterpret12/1 -> out12/1
  slice12/1 -> reinterpret12/1
  reinterpret13/1 -> out13/1
  slice13/1 -> reinterpret13/1
  reinterpret14/1 -> out14/1
  slice14/1 -> reinterpret14/1
  reinterpret15/1 -> out15/1
  slice15/1 -> reinterpret15/1
  reinterpret16/1 -> out16/1
  slice16/1 -> reinterpret16/1
  reinterpret17/1 -> out17/1
  slice17/1 -> reinterpret17/1
  reinterpret18/1 -> out18/1
  slice18/1 -> reinterpret18/1
  reinterpret19/1 -> out19/1
  slice19/1 -> reinterpret19/1
  reinterpret20/1 -> out20/1
  slice20/1 -> reinterpret20/1
  reinterpret21/1 -> out21/1
  slice21/1 -> reinterpret21/1
  reinterpret22/1 -> out22/1
  slice22/1 -> reinterpret22/1
  reinterpret23/1 -> out23/1
  slice23/1 -> reinterpret23/1
  reinterpret24/1 -> out24/1
  slice24/1 -> reinterpret24/1
  reinterpret25/1 -> out25/1
  slice25/1 -> reinterpret25/1
  reinterpret26/1 -> out26/1
  slice26/1 -> reinterpret26/1
  reinterpret27/1 -> out27/1
  slice27/1 -> reinterpret27/1
  reinterpret28/1 -> out28/1
  slice28/1 -> reinterpret28/1
  reinterpret29/1 -> out29/1
  slice29/1 -> reinterpret29/1
  reinterpret30/1 -> out30/1
  slice30/1 -> reinterpret30/1
  reinterpret31/1 -> out31/1
  slice31/1 -> reinterpret31/1
  reinterpret32/1 -> out32/1
  slice32/1 -> reinterpret32/1
  reinterpret33/1 -> out33/1
  slice33/1 -> reinterpret33/1
  reinterpret34/1 -> out34/1
  slice34/1 -> reinterpret34/1
  reinterpret35/1 -> out35/1
  slice35/1 -> reinterpret35/1
  reinterpret36/1 -> out36/1
  slice36/1 -> reinterpret36/1
  reinterpret37/1 -> out37/1
  slice37/1 -> reinterpret37/1
  reinterpret38/1 -> out38/1
  slice38/1 -> reinterpret38/1
  reinterpret39/1 -> out39/1
  slice39/1 -> reinterpret39/1
  reinterpret40/1 -> out40/1
  slice40/1 -> reinterpret40/1
  reinterpret41/1 -> out41/1
  slice41/1 -> reinterpret41/1
  reinterpret42/1 -> out42/1
  slice42/1 -> reinterpret42/1
  reinterpret43/1 -> out43/1
  slice43/1 -> reinterpret43/1
  reinterpret44/1 -> out44/1
  slice44/1 -> reinterpret44/1
  reinterpret45/1 -> out45/1
  slice45/1 -> reinterpret45/1
  reinterpret46/1 -> out46/1
  slice46/1 -> reinterpret46/1
  reinterpret47/1 -> out47/1
  slice47/1 -> reinterpret47/1
  reinterpret48/1 -> out48/1
  slice48/1 -> reinterpret48/1
  reinterpret49/1 -> out49/1
  slice49/1 -> reinterpret49/1
  reinterpret50/1 -> out50/1
  slice50/1 -> reinterpret50/1
  reinterpret51/1 -> out51/1
  slice51/1 -> reinterpret51/1
  reinterpret52/1 -> out52/1
  slice52/1 -> reinterpret52/1
  reinterpret53/1 -> out53/1
  slice53/1 -> reinterpret53/1
  reinterpret54/1 -> out54/1
  slice54/1 -> reinterpret54/1
  reinterpret55/1 -> out55/1
  slice55/1 -> reinterpret55/1
  reinterpret56/1 -> out56/1
  slice56/1 -> reinterpret56/1
  reinterpret57/1 -> out57/1
  slice57/1 -> reinterpret57/1
  reinterpret58/1 -> out58/1
  slice58/1 -> reinterpret58/1
  reinterpret59/1 -> out59/1
  slice59/1 -> reinterpret59/1
  reinterpret60/1 -> out60/1
  slice60/1 -> reinterpret60/1
  reinterpret61/1 -> out61/1
  slice61/1 -> reinterpret61/1
  reinterpret62/1 -> out62/1
  slice62/1 -> reinterpret62/1
  reinterpret63/1 -> out63/1
  slice63/1 -> reinterpret63/1
  reinterpret64/1 -> out64/1
  slice64/1 -> reinterpret64/1
  reinterpret65/1 -> out65/1
  slice65/1 -> reinterpret65/1
  reinterpret66/1 -> out66/1
  slice66/1 -> reinterpret66/1
  reinterpret67/1 -> out67/1
  slice67/1 -> reinterpret67/1
  reinterpret68/1 -> out68/1
  slice68/1 -> reinterpret68/1
  reinterpret69/1 -> out69/1
  slice69/1 -> reinterpret69/1
  reinterpret70/1 -> out70/1
  slice70/1 -> reinterpret70/1
  reinterpret71/1 -> msb_out71/1
  slice71/1 -> reinterpret71/1
  bus_in/1 -> slice1/1, slice2/1, slice3/1, slice4/1, slice5/1, slice6/1, slice7/1, slice8/1, slice9/1, slice10/1, slice11/1, slice12/1, slice13/1, slice14/1, slice15/1, slice16/1, slice17/1, slice18/1, slice19/1, slice20/1, slice21/1, slice22/1, slice23/1, slice24/1, slice25/1, slice26/1, slice27/1, slice28/1, slice29/1, slice30/1, slice31/1, slice32/1, slice33/1, slice34/1, slice35/1, slice36/1, slice37/1, slice38/1, slice39/1, slice40/1, slice41/1, slice42/1, slice43/1, slice44/1, slice45/1, slice46/1, slice47/1, slice48/1, slice49/1, slice50/1, slice51/1, slice52/1, slice53/1, slice54/1, slice55/1, slice56/1, slice57/1, slice58/1, slice59/1, slice60/1, slice61/1, slice62/1, slice63/1, slice64/1, slice65/1, slice66/1, slice67/1, slice68/1, slice69/1, slice70/1, slice71/1

== system r2_b8a4x1kf/sys1/vacc_tvg0/ins_counter/bus_replicate1/bussify ==
  in1 : Inport
  in2 : Inport  Port=2
  concatenate : xbsIndex_r4/Concat  num_inputs=2  dbl_ovrd=off  block_type=concat
  reinterpret1 : xbsIndex_r4/Reinterpret  force_arith_type=on  arith_type=Unsigned  force_bin_pt=on  bin_pt=0  block_type=reinterpret
      settings: infoedit="Changes signal type without altering the binary representation.   You can changed the signal between signed and unsigned, and relocate the binary point.<br><br>Hardware notes: In hardware this block costs nothing.<br><br>Example:  Suppose the input is 6 bits wide, signed, with 2 fractional bits, and the output is forced to unsigned with 0 fractional bits.  Then an input of -2.0 (1110.00 in binary 2's complement) becomes an output of 56 (111000 in binary)."
  reinterpret2 : xbsIndex_r4/Reinterpret  force_arith_type=on  arith_type=Unsigned  force_bin_pt=on  bin_pt=0  block_type=reinterpret
      settings: infoedit="Changes signal type without altering the binary representation.   You can changed the signal between signed and unsigned, and relocate the binary point.<br><br>Hardware notes: In hardware this block costs nothing.<br><br>Example:  Suppose the input is 6 bits wide, signed, with 2 fractional bits, and the output is forced to unsigned with 0 fractional bits.  Then an input of -2.0 (1110.00 in binary 2's complement) becomes an output of 56 (111000 in binary)."
  bus_out : Outport
  wires:
  reinterpret2/1 -> concatenate/2
  in2/1 -> reinterpret2/1
  reinterpret1/1 -> concatenate/1
  in1/1 -> reinterpret1/1
  concatenate/1 -> bus_out/1

== system r2_b8a4x1kf/sys1/xeng/auto_tap/dual_pol_cmac/cmac1 ==
  a+bi : Inport
  c+di : Inport  Port=2
  acc_in : Inport  Port=3
  sync : Inport  Port=4
  valid_in : Inport  Port=5
  Constant1 : xbsIndex_r4/Constant  const=0  gui_display_data_type=Fixed-point  arith_type=Unsigned  n_bits=bit_growth  bin_pt=0  preci_type=Single  exp_width=8  frac_width=24  explicit_period=on  period=1  equ=P=C  opselect=C  inp2=PCIN>>17  opr=+  inp1=P  carry=CIN  dbl_ovrd=off  block_type=constant
      settings: block_version=9.2.01
  Constant2 : xbsIndex_r4/Constant  const=0  gui_display_data_type=Fixed-point  arith_type=Unsigned  n_bits=1  bin_pt=0  preci_type=Single  exp_width=8  frac_width=24  explicit_period=on  period=1  equ=P=C  opselect=C  inp2=PCIN>>17  opr=+  inp1=P  carry=CIN  dbl_ovrd=off  block_type=constant
      settings: block_version=9.2.01
  Counter : xbsIndex_r4/Counter  cnt_type=Count Limited  cnt_to=acc_len - 1  operation=Up  start_count=0  cnt_by_val=1  arith_type=Unsigned  n_bits=bit_growth  bin_pt=0  load_pin=off  rst=on  en=off  explicit_period=off  period=1  dbl_ovrd=off  use_behavioral_HDL=off  implementation=Fabric  use_rpm=on  block_type=counter
      settings: xl_area=[0, 0, 0, 0, 0, 0, 0]  block_version=9.2.01
  Delay : xbsIndex_r4/Delay  rst=off  infoeditControl=Selection of Reset will increase slice count due to use of real FFs and instead of SRLs  en=off  latency=add_latency + mult_latency - 1  dbl_ovrd=off  reg_retiming=on  block_type=delay
      settings: xl_area=[0, 0, 0, 0, 0, 0, 0]  block_version=9.2.01
  Relational : xbsIndex_r4/Relational  mode=a=b  en=off  latency=1  dbl_ovrd=off  block_type=relational
      settings: xl_area=[0, 0, 0, 0, 0, 0, 0]  block_version=9.2.01
  Terminator : Terminator
  acc : Subsystem
  acc1 : Subsystem
  c_to_ri1 : Subsystem
  c_to_ri2 : Subsystem
  cmult* : Subsystem  AncestorBlock=casper_library_multipliers/cmult  mask(cmult){n_bits_a=8, bin_pt_a=7, n_bits_b=8, bin_pt_b=7, n_bits_ab=25, bin_pt_ab=14, quantization=Truncate, overflow=Wrap, in_latency=0, mult_latency=4, add_latency=3, conv_latency=0, conjugated=on, async=off, pipelined_enable=on, multiplier_implementation=embedded multiplier core}
      mask prompts: n_bits_a "Number of Bits 'a'"; bin_pt_a "Binary Point 'a'"; n_bits_b "Number of Bits 'b'"; bin_pt_b "Binary Point 'b'"; n_bits_ab "Number of Bits 'ab'"; bin_pt_ab "Binary Point 'ab'"; in_latency "Input latency"; mult_latency "Multiplier Latency"; add_latency "Adder Latency"; conv_latency "Convert latency"; conjugated "Conjugate"; async "asynchronous operation"; pipelined_enable "enable pipeline"; multiplier_implementation "Multiplier implementation"
      mask help:
      | Multiplies two complex numbers using 4 multipliers and 2 adders.
      | Conjugation is optional.
      mask init: same as r2_b8a4x1kf/sys0/xeng/auto_tap/dual_pol_cmac/cmac1/cmult*
      settings: AttributesFormatString=|
      | 8_7 * 8_7 ==> 25_14
      | Truncate, Wrap
      | Latency=0
      mask TypeOptions quantization: Truncate | Round  (unbiased: +/- Inf) | Round  (unbiased: Even Values)
      mask TypeOptions overflow: Wrap | Saturate | Flag as error
      mask TypeOptions multiplier_implementation: behavioral HDL | standard core | embedded multiplier core
  ri_to_c : Subsystem
  acc_out : Outport
  valid_out : Outport  Port=2
  wires:
  cmult*/1(ab) -> c_to_ri1/1(In1)
  valid_in/1 -> acc1/4(valid_in)
  acc1/2(valid_out) -> valid_out/1
  acc/2(valid_out) -> Terminator/1
  Constant2/1 -> acc/4(valid_in)
  Delay/1 -> Counter/1
  sync/1 -> Delay/1
  Constant1/1 -> Relational/2
  Counter/1 -> Relational/1
  Relational/1 -> acc1/1(rst), acc/1(rst)
  c_to_ri2/2(Out2) -> acc1/3(acc_in)
  ri_to_c/1(Out1) -> acc_out/1
  acc1/1(acc_out) -> ri_to_c/2(In2)
  acc_in/1 -> c_to_ri2/1(In1)
  c+di/1 -> cmult*/2(b)
  a+bi/1 -> cmult*/1(a)
  c_to_ri1/1(Out1) -> acc/2(din)  "auto_real"
  c_to_ri1/2(Out2) -> acc1/2(din)
  acc/1(acc_out) -> ri_to_c/1(In1)
  c_to_ri2/1(Out1) -> acc/3(acc_in)
